simulink model "mo_hinh_dwt_wiener"  (R2026b)
settings: Solver=FixedStepDiscrete  StopTime=5.2480000000000002  FixedStep=6.2500000000000001e-05
InitFcn:
  | model = bdroot;
  | roleMatches=find_system(model,'LookUnderMasks','all','FollowLinks','off','IncludeCommented','on','Tag','WaveletDSP:source');
  | assert(numel(roleMatches)==1,'WaveletDSP:Role','Thiếu hoặc trùng định danh nội bộ: source. Không cần khôi phục tên hiển thị.');
  | source=get_param(roleMatches{1},'Handle');
  | roleMatches=find_system(model,'LookUnderMasks','all','FollowLinks','off','IncludeCommented','on','Tag','WaveletDSP:clean');
  | assert(numel(roleMatches)==1,'WaveletDSP:Role','Thiếu hoặc trùng định danh nội bộ: clean. Không cần khôi phục tên hiển thị.');
  | cleanSource=get_param(roleMatches{1},'Handle');
  | roleMatches=find_system(model,'LookUnderMasks','all','FollowLinks','off','IncludeCommented','on','Tag','WaveletDSP:sink');
  | assert(numel(roleMatches)==1,'WaveletDSP:Role','Thiếu hoặc trùng định danh nội bộ: sink. Không cần khôi phục tên hiển thị.');
  | sink=get_param(roleMatches{1},'Handle');
  | roleMatches=find_system(model,'LookUnderMasks','all','FollowLinks','off','IncludeCommented','on','Tag','WaveletDSP:filter');
  | assert(numel(roleMatches)==1,'WaveletDSP:Role','Thiếu hoặc trùng định danh nội bộ: filter. Không cần khôi phục tên hiển thị.');
  | filterBlock=get_param(roleMatches{1},'Handle');
  | roleMatches=find_system(model,'LookUnderMasks','all','FollowLinks','off','IncludeCommented','on','Tag','WaveletDSP:reference_sync');
  | assert(numel(roleMatches)==1,'WaveletDSP:Role','Thiếu hoặc trùng định danh nội bộ: reference_sync. Không cần khôi phục tên hiển thị.');
  | referenceSync=get_param(roleMatches{1},'Handle');
  | roleMatches=find_system(model,'LookUnderMasks','all','FollowLinks','off','IncludeCommented','on','Tag','WaveletDSP:noisy_sync');
  | assert(numel(roleMatches)==1,'WaveletDSP:Role','Thiếu hoặc trùng định danh nội bộ: noisy_sync. Không cần khôi phục tên hiển thị.');
  | noisySync=get_param(roleMatches{1},'Handle');
  | workspace = get_param(model,'ModelWorkspace');
  | assignin(workspace,'Export_Complete',false);
  | inputFile = get_param(source,'inputFilename');
  | inputInfo = audioinfo(inputFile);
  | assert(inputInfo.NumChannels==1,'Chỉ hỗ trợ âm thanh một kênh.');
  | useClean = strcmp(get_param(filterBlock,'Use_Clean'),'1');
  | cleanFile = get_param(cleanSource,'inputFilename');
  | if useClean && strcmp(get_param(filterBlock,'Auto_Clean'),'1')
  |     [inputFolder,inputStem] = fileparts(inputFile);
  |     recordId = regexp(inputStem,'^(speech_\d+)_','tokens','once');
  |     assert(~isempty(recordId),'Không tìm được âm thanh sạch; tắt ghép tệp tự động và chọn tệp tham chiếu trực tiếp.');
  |     cleanFile = fullfile(fileparts(fileparts(inputFolder)),'clean',[recordId{1} '.wav']);
  | end
  | frameSize = str2double(get_param(source,'SamplesPerFrame'));
  | assert(isfinite(frameSize) && frameSize>0 && mod(frameSize,128)==0,'Số mẫu mỗi khung âm thanh có nhiễu phải là bội dương của 128.');
  | if useClean
  |     cleanInfo = audioinfo(cleanFile);
  |     assert(cleanInfo.SampleRate==inputInfo.SampleRate && cleanInfo.TotalSamples==inputInfo.TotalSamples && cleanInfo.NumChannels==1,'Âm thanh sạch/noisy must match sample rate and length.');
  |     if ~strcmp(get_param(filterBlock,'Auto_Frame'),'1')
  |         assert(str2double(get_param(cleanSource,'SamplesPerFrame'))==frameSize,'Âm thanh sạch/Noisy frame sizes differ. Set them explicitly or enable Auto_Frame.');
  |     end
  | end
  | levels = [1 2 3 4 5 6 7 7];
  | powerWindow = str2double(get_param(filterBlock,'Win_Pow'));
  | smoothWindow = str2double(get_param(filterBlock,'Win_Smooth'));
  | powerLengths = max(1,round(powerWindow*inputInfo.SampleRate./2.^levels));
  | smoothLengths = max(1,round(smoothWindow*inputInfo.SampleRate./2.^levels));
  | bandDelays = floor((powerLengths-1)/2)+floor((smoothLengths-1)/2);
  | totalDelay = 29*(2^7-1)+128*ceil(max(bandDelays.*2.^levels)/128);
  | frameCount = ceil((inputInfo.TotalSamples+totalDelay)/frameSize);
  | requiredStop = (frameCount-1)*frameSize/inputInfo.SampleRate;
  | autoRun = strcmp(get_param(filterBlock,'Auto_Run'),'1');
  | if ~autoRun
  |     assert(strcmp(get_param(model,'Solver'),'FixedStepDiscrete'),'Chọn bộ giải rời rạc bước cố định hoặc bật tự tính thời gian mô phỏng.');
  |     stepValue = slResolve(get_param(model,'FixedStep'),model);
  |     stopValue = slResolve(get_param(model,'StopTime'),model);
  |     assert(isscalar(stepValue) && isfinite(stepValue) && stepValue>0 && stepValue<=1/inputInfo.SampleRate && abs((1/inputInfo.SampleRate)/stepValue-round((1/inputInfo.SampleRate)/stepValue))<1e-8,'Bước mô phỏng phải chia hết chu kỳ lấy mẫu; chỉnh bước hoặc bật tự tính thời gian.');
  |     assert(isscalar(stopValue) && isfinite(stopValue) && stopValue>=requiredStop,'Thời gian dừng quá ngắn hoặc vô hạn; đặt thời gian hữu hạn đủ dài hoặc bật tự tính thời gian.');
  | end
  | configuredOutput = get_param(sink,'outputFilename');
  | assert(~strcmp(inputFile,configuredOutput) && ~strcmp(cleanFile,configuredOutput),'Tệp đầu ra không được trùng tệp đầu vào.');
  | [outputFolder,outputStem,outputExtension] = fileparts(configuredOutput);
  | if isempty(outputFolder), outputFolder=pwd; end
  | if ~isfolder(outputFolder), mkdir(outputFolder); end
  | runtimeOutput = configuredOutput;
  | if isfile(runtimeOutput)
  |     runtimeOutput = fullfile(outputFolder,[outputStem '_' char(datetime('now','Format','yyyyMMdd_HHmmss_SSS')) outputExtension]);
  |     assert(~isfile(runtimeOutput),'Trùng tên tệp đầu ra; chọn tên khác và chạy lại.');
  | end
  | restoreSettings = struct('CleanFile',get_param(cleanSource,'inputFilename'),'CleanFrame',get_param(cleanSource,'SamplesPerFrame'),'CleanCommented',get_param(cleanSource,'Commented'),'OutputFile',configuredOutput,'SolverType',get_param(model,'SolverType'),'Solver',get_param(model,'Solver'),'FixedStep',get_param(model,'FixedStep'),'StopTime',get_param(model,'StopTime'));
  | assignin(workspace,'Run_Restore_Settings',restoreSettings);
  | assignin(workspace,'Last_Output_File',runtimeOutput);
  | assignin(workspace,'Total_Delay',totalDelay);
  | for syncBlock=[referenceSync noisySync]
  |     countText=sprintf('%.0f',totalDelay);
  |     if ~strcmp(get_param(syncBlock,'Sample_Count'),countText), set_param(syncBlock,'Sample_Count',countText); end
  | end
  | assignin(workspace,'Valid_Samples',inputInfo.TotalSamples);
  | assignin(workspace,'Audio_Fs',inputInfo.SampleRate);
  | assignin(workspace,'Frame_Size',frameSize);
  | assignin(workspace,'Reference_Available',double(useClean));
  | assignin(workspace,'Run_Clean_File',cleanFile);
  | if useClean
  |     set_param(cleanSource,'inputFilename',cleanFile,'Commented','off');
  |     referenceSource = cleanSource;
  | else
  |     set_param(cleanSource,'inputFilename',inputFile,'Commented','on');
  |     referenceSource = source;
  | end
  | if strcmp(get_param(filterBlock,'Auto_Frame'),'1'), set_param(cleanSource,'SamplesPerFrame',num2str(frameSize)); end
  | referencePorts = get_param(referenceSync,'PortHandles');
  | referenceLine = get_param(referencePorts.Inport(1),'Line');
  | if referenceLine~=-1
  |     oldSource = get_param(get_param(get_param(referenceLine,'SrcPortHandle'),'Parent'),'Handle');
  |     if oldSource~=referenceSource
  |         delete_line(referenceLine);
  |         sourcePorts=get_param(referenceSource,'PortHandles');
  |         add_line(model,sourcePorts.Outport(1),referencePorts.Inport(1),'autorouting','on');
  |     end
  | else
  |     sourcePorts=get_param(referenceSource,'PortHandles');
  |     add_line(model,sourcePorts.Outport(1),referencePorts.Inport(1),'autorouting','on');
  | end
  | if autoRun
  |     set_param(model,'SolverType','Fixed-step','Solver','FixedStepDiscrete','FixedStep',sprintf('%.17g',1/inputInfo.SampleRate),'StopTime',sprintf('%.17g',requiredStop));
  | end
  | set_param(sink,'outputFilename',runtimeOutput);
  | fprintf('Có tham chiếu=%d. Tệp đầu ra thực tế: %s\n',useClean,runtimeOutput);
StopFcn:
  | model = bdroot;
  | workspace = get_param(model,'ModelWorkspace');
  | roleMatches=find_system(model,'LookUnderMasks','all','FollowLinks','off','IncludeCommented','on','Tag','WaveletDSP:sink');
  | assert(numel(roleMatches)==1,'WaveletDSP:Role','Thiếu hoặc trùng định danh nội bộ: sink. Không cần khôi phục tên hiển thị.');
  | sink=get_param(roleMatches{1},'Handle');
  | roleMatches=find_system(model,'LookUnderMasks','all','FollowLinks','off','IncludeCommented','on','Tag','WaveletDSP:clean');
  | assert(numel(roleMatches)==1,'WaveletDSP:Role','Thiếu hoặc trùng định danh nội bộ: clean. Không cần khôi phục tên hiển thị.');
  | cleanSource=get_param(roleMatches{1},'Handle');
  | outputFile = evalin(workspace,'Last_Output_File');
  | restoreSettings = evalin(workspace,'Run_Restore_Settings');
  | set_param(sink,'outputFilename',restoreSettings.OutputFile);
  | set_param(cleanSource,'inputFilename',restoreSettings.CleanFile,'Commented',restoreSettings.CleanCommented);
  | [outputAudio,outputRate] = audioread(outputFile);
  | delaySamples = evalin(workspace,'Total_Delay');
  | validSamples = evalin(workspace,'Valid_Samples');
  | assert(size(outputAudio,1)>=delaySamples+validSamples,'Mô phỏng dừng sớm: đầu ra chưa đủ mẫu; tệp thô được giữ lại.');
  | outputAudio = outputAudio(delaySamples+(1:validSamples),:);
  | audiowrite(outputFile,outputAudio,outputRate,'BitsPerSample',24);
  | assignin(workspace,'Export_Complete',true);
  | fprintf('Đã xuất âm thanh và giữ thiết lập. Tệp âm thanh: %s\n',outputFile);
model workspace (MAT data in the model file):
  Audio_Fs = 16000
  Export_Complete = 1
  Frame_Size = 1024
  Last_Output_File = '/home/alberttochiro/Documents/Codex/PRJ/WaveletDSP/results/denoised_output_20261108_091202_407.wav'
  Reference_Available = 1
  Run_Clean_File = '/home/alberttochiro/Documents/Codex/PRJ/WaveletDSP/data_DSP_speech/clean/speech_004.wav'
  Run_Restore_Settings.CleanFile = '/home/alberttochiro/Documents/Codex/PRJ/WaveletDSP/data_DSP_speech/clean/speech_004.wav'
  Run_Restore_Settings.CleanFrame = '1024'
  Run_Restore_Settings.CleanCommented = 'off'
  Run_Restore_Settings.OutputFile = '/home/alberttochiro/Documents/Codex/PRJ/WaveletDSP/results/denoised_output.wav'
  Run_Restore_Settings.SolverType = 'Fixed-step'
  Run_Restore_Settings.Solver = 'FixedStepDiscrete'
  Run_Restore_Settings.FixedStep = '6.2500000000000001e-05'
  Run_Restore_Settings.StopTime = '5.2480000000000002'
  Total_Delay = 4579
  Valid_Samples = 79500
undefined symbols (not defined in the file or in its folder): dspblkCoreblockFVToolHelper, gcbh, Pn_1, Pn_2, Pn_3, Pn_4, Pn_5, Pn_6, Pn_7, Pn_8
libraries: dspvision x3, dspmlti4 x2, simulink x2
(part 1 of 2)
settings Model: Creator=alberttochiro  LastModifiedBy=alberttochiro

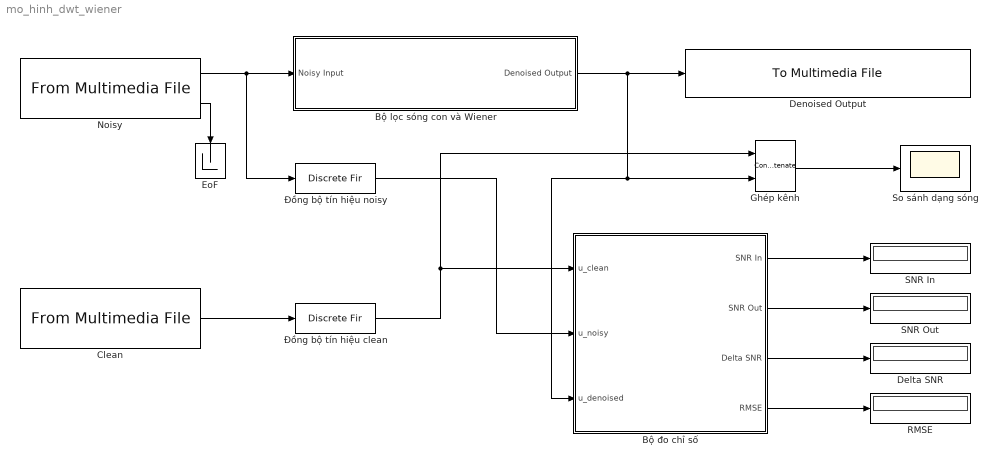
== system mo_hinh_dwt_wiener ==
  Bộ lọc sóng con và Wiener : Subsystem  Tag=WaveletDSP:filter  mask(Bo Loc Wavelet DWT Wiener Full Native){Noise_Sec=0.25, Win_Pow=0.064, Win_Smooth=0.040, Gain_Floor=0.05, Auto_Clean=1, Noise_Auto=1, Noise_Powers=[0.000004 0.000008 0.000014 0.000025 0.000055 0.000108 0.000112 0.002000], Use_Clean=1, Clean_File=/home/alberttochiro/Documents/Codex/PRJ/WaveletDSP/data_DSP_speech/clean/speech_003.wav, Noise_Start_Auto=1, Noise_Start=0, Auto_Run=0, Auto_Frame=0, Noise_Power_1=4e-06, Noise_Power_2=8e-06, Noise_Power_3=1.4e-05, Noise_Power_4=2.5e-05, Noise_Power_5=5.5e-05, Noise_Power_6=0.000108, Noise_Power_7=0.000112, Noise_Power_8=0.002}
      mask prompts: Noise_Sec "Độ dài mẫu nhiễu (giây)"; Win_Pow "Cửa sổ tính công suất (giây)"; Win_Smooth "Cửa sổ làm mượt hệ số khuếch đại (giây)"; Gain_Floor "Hệ số khuếch đại tối thiểu (từ 0 đến 1)"; Auto_Clean "Tự ghép tệp âm thanh sạch cùng bản ghi (1 là bật, 0 là tắt)"; Noise_Auto "Tự ước lượng công suất nhiễu (1 là bật, 0 là nhập tay)"; Noise_Powers "Công suất nhiễu tám dải khi nhập tay"; Use_Clean "Dùng âm thanh sạch để đánh giá (1 là có, 0 là không)"; Clean_File "Đường dẫn tham chiếu cũ (không sử dụng)"; Noise_Start_Auto "Tự bỏ đoạn đầu hằng khi lấy mẫu nhiễu (1 là tự động, 0 là chọn tay)"; Noise_Start "Thời điểm bắt đầu lấy mẫu nhiễu thủ công (giây)"; Auto_Run "Tự tính bước và thời gian mô phỏng (1 là bật, 0 là giữ thiết lập)"; Auto_Frame "Tự đồng bộ kích thước khung tham chiếu (1 là bật, 0 là kiểm tra)"; Noise_Power_1 "Công suất nhiễu dải 1 khi nhập tay"; Noise_Power_2 "Công suất nhiễu dải 2 khi nhập tay"; Noise_Power_3 "Công suất nhiễu dải 3 khi nhập tay"; Noise_Power_4 "Công suất nhiễu dải 4 khi nhập tay"; Noise_Power_5 "Công suất nhiễu dải 5 khi nhập tay"; Noise_Power_6 "Công suất nhiễu dải 6 khi nhập tay"; Noise_Power_7 "Công suất nhiễu dải 7 khi nhập tay"; Noise_Power_8 "Công suất nhiễu dải 8 khi nhập tay"
      mask help:
      | Bộ lọc phân rã sóng con bảy mức kết hợp Wiener.
      | Các khối xử lý tín hiệu giữ nguyên công thức. Ước lượng nhiễu vẫn nằm trong phần khởi tạo mặt nạ.
      | Không cần chạy tệp lệnh bên ngoài. Đoạn lấy mẫu nhiễu phải chỉ chứa tiếng nền, không có lời nói.
      mask init:
      | validateattributes(Noise_Power_1,{'double'},{'scalar','real','finite','nonnegative'});
      | validateattributes(Noise_Power_2,{'double'},{'scalar','real','finite','nonnegative'});
      | validateattributes(Noise_Power_3,{'double'},{'scalar','real','finite','nonnegative'});
      | validateattributes(Noise_Power_4,{'double'},{'scalar','real','finite','nonnegative'});
      | validateattributes(Noise_Power_5,{'double'},{'scalar','real','finite','nonnegative'});
      | validateattributes(Noise_Power_6,{'double'},{'scalar','real','finite','nonnegative'});
      | validateattributes(Noise_Power_7,{'double'},{'scalar','real','finite','nonnegative'});
      | validateattributes(Noise_Power_8,{'double'},{'scalar','real','finite','nonnegative'});
      | roleMatches=find_system(bdroot,'LookUnderMasks','all','FollowLinks','off','IncludeCommented','on','Tag','WaveletDSP:source');
      | assert(numel(roleMatches)==1,'WaveletDSP:Role','Thiếu hoặc trùng định danh nội bộ: source. Không cần khôi phục tên hiển thị.');
      | audioSource=get_param(roleMatches{1},'Handle');
      | inFile = get_param(audioSource,'inputFilename');
      | inputInfo = audioinfo(inFile);
      | Fs = inputInfo.SampleRate;
      | validateattributes(Win_Pow, {'double'}, {'scalar','positive','finite'});
      | validateattributes(Win_Smooth, {'double'}, {'scalar','positive','finite'});
      | validateattributes(Gain_Floor, {'double'}, {'scalar','>=',0,'<=',1});
      | wname = 'coif5';
      | lev = 7;
      | if Noise_Auto == 1
      |         [x_calib, Fs_calib] = audioread(inFile);
      | validateattributes(Noise_Sec,{'double'},{'scalar','real','finite','positive'});
      | validateattributes(Noise_Start,{'double'},{'scalar','real','finite','nonnegative'});
      | validateattributes(Noise_Start_Auto,{'double'},{'scalar','binary'});
      | assert(size(x_calib,2)==1 && all(isfinite(x_calib(:))), 'WaveletDSP:InvalidNoiseProfile', 'Mẫu nhiễu cần âm thanh một kênh có giá trị hữu hạn.');
      | N_n = floor(Noise_Sec*Fs_calib);
      | Startup_Skipped_Samples = 0;
      | if Noise_Start_Auto==1
      |     firstChanged = find(x_calib~=x_calib(1),1,'first');
      |     assert(~isempty(firstChanged), 'WaveletDSP:ConstantRecording', 'Toàn bộ bản ghi có giá trị hằng. Hãy ghi tiếng nền trước khi nói hoặc nhập công suất nhiễu thủ công.');
      |     if firstChanged-1>=ceil(0.010*Fs_calib)
      |         Startup_Skipped_Samples = firstChanged-1;
      |     end
      |     Noise_Profile_Start_Sample = Startup_Skipped_Samples+1;
      | else
      |     Noise_Profile_Start_Sample = floor(Noise_Start*Fs_calib)+1;
      | end
      | Noise_Profile_End_Sample = Noise_Profile_Start_Sample+N_n-1;
      | assert(N_n>=1024 && Noise_Profile_End_Sample<=numel(x_calib), 'WaveletDSP:InvalidNoiseProfile', 'Mẫu nhiễu cần ít nhất 1024 mẫu và không vượt cuối tệp; giảm độ dài hoặc chọn lại thời điểm bắt đầu.');
      | noiseProfile = x_calib(Noise_Profile_Start_Sample:Noise_Profile_End_Sample);
      | assert(var(noiseProfile,1)>eps(max(abs(noiseProfile)))^2, 'WaveletDSP:ConstantNoiseProfile', 'Mẫu nhiễu được chọn có giá trị hằng hoặc gần hằng ở mức sai số số học. Bật tự bỏ đoạn đầu hằng hoặc chọn lại đoạn chỉ có tiếng nền.');
      | fprintf('Mẫu nhiễu: bắt đầu=%.9f giây, độ dài=%.9f giây, bỏ đoạn đầu hằng=%d mẫu. Chức năng này không phát hiện tiếng nói.\n', (Noise_Profile_Start_Sample-1)/Fs_calib,N_n/Fs_calib,Startup_Skipped_Samples);
      | [C_n, L_n] = wavedec(noiseProfile, lev, wname, 'Mode', 'sym');
      | Pn_vec = zeros(1, 8);
      |         for k = 1:7
      |             Pn_vec(k) = var(detcoef(C_n, L_n, k), 1);
      |         end
      |         Pn_vec(8) = var(appcoef(C_n, L_n, wname, 7), 1);
      | else
      |     Pn_vec = [Noise_Power_1 Noise_Power_2 Noise_Power_3 Noise_Power_4 Noise_Power_5 Noise_Power_6 Noise_Power_7 Noise_Power_8];
      | end
      | validateattributes(Pn_vec, {'double'}, {'vector','numel',8,'nonnegative','finite'});
      | levels = [1, 2, 3, 4, 5, 6, 7, 7];
      | delays_tree = [1827, 899, 435, 203, 87, 29, 0, 0];
      | window_power = max(1, round(Win_Pow*Fs./2.^levels));
      | window_smooth = max(1, round(Win_Smooth*Fs./2.^levels));
      | sync_delays = floor((window_power-1)/2)+floor((window_smooth-1)/2);
      | common_delay = 128*ceil(max(sync_delays.*2.^levels)/128);
      | delays_tree = delays_tree+(common_delay-sync_delays.*2.^levels)./2.^levels;
      | for k = 1:8
      |     Fs_k = Fs / (2^levels(k));
      |     w_pow_k = max(1, round(Win_Pow * Fs_k));
      |     w_sm_k = max(1, round(Win_Smooth * Fs_k));
      |     d_sync_k = floor((w_pow_k - 1)/2) + floor((w_sm_k - 1)/2);
      |     eval(sprintf('b_pow_%d = ones(1, %d)/%d;', k, w_pow_k, w_pow_k));
      |     eval(sprintf('b_sm_%d = ones(1, %d)/%d;', k, w_sm_k, w_sm_k));
      |     eval(sprintf('b_sync_%d = [zeros(1, %d), 1];', k, d_sync_k));
      |     eval(sprintf('b_tree_%d = [zeros(1, %d), 1];', k, delays_tree(k)));
      |     eval(sprintf('Pn_%d = %.12e;', k, Pn_vec(k)));
      | end
      | 
      | numericInterfaceVersion='WaveletDSP:NumericInterface';
      | for bandIndex=1:8
      |     counts=[sync_delays(bandIndex) window_power(bandIndex) window_smooth(bandIndex) delays_tree(bandIndex)];
      |     kinds={'sync','pow','sm','tree'};
      |     for kindIndex=1:4
      |         roleName=sprintf('WaveletDSP:%s_%d',kinds{kindIndex},bandIndex);
      |         matches=find_system(bdroot,'LookUnderMasks','all','FollowLinks','off','IncludeCommented','on','Tag',roleName);
      |         assert(numel(matches)==1,'WaveletDSP:Role','Thiếu hoặc trùng định danh nội bộ: %s.',roleName);
      |         countText=sprintf('%.0f',counts(kindIndex));
      |         if ~strcmp(get_param(matches{1},'Sample_Count'),countText), set_param(matches{1},'Sample_Count',countText); end
      |     end
      | end
  Bộ đo chỉ số : Subsystem
  Clean : dspvision/From Multimedia File  Tag=WaveletDSP:clean  inputFilename=/home/alberttochiro/Documents/Codex/PRJ/WaveletDSP/data_DSP_speech/clean/speech_004.wav  readRange=[1 Inf]  loop=on  numPlays=1  outputStreams=Audio only  videoDataType=single  audioDataType=double  inheritSampleTime=on  userDefinedSampleTime=1/30  noAudioOutput=off  isIntensityVideo=off  fourcc=RGB  colorVideoFormat=One multidimensional signal  outputEOF=off  dataOrg=Column-major  audioFrameSize=1024  computeAudioFrameSize=off  outSamplingMode=Sample based
      settings: LibrarySourceBlock=dspsrcs4/From Multimedia File
  Delta SNR : Display
  Denoised Output : dspvision/To Multimedia File  Tag=WaveletDSP:sink  outputFilename=/home/alberttochiro/Documents/Codex/PRJ/WaveletDSP/results/denoised_output.wav  streamSelection=Audio only  videoCompressor=None (uncompressed)  audioCompressor=None (uncompressed)  imagePorts=One multidimensional signal  fileType=WAV  audioDatatype=24-bit integer  fourcc=RGB  audioBitRate=128  audioQuality=75  videoQuality=75  mj2000CompFactor=10
  EoF : Terminator
  Ghép kênh : Concatenate  Mode=Multidimensional array  ConcatenateDimension=2
  Noisy : dspvision/From Multimedia File  Tag=WaveletDSP:source  inputFilename=/home/alberttochiro/Documents/Codex/PRJ/WaveletDSP/data_DSP_speech/noisy/white_10db/speech_004_white_10dB.wav  readRange=[1 Inf]  loop=on  numPlays=1  outputStreams=Audio only  videoDataType=single  audioDataType=double  inheritSampleTime=on  userDefinedSampleTime=1/30  noAudioOutput=off  isIntensityVideo=off  fourcc=RGB  colorVideoFormat=One multidimensional signal  outputEOF=on  dataOrg=Column-major  audioFrameSize=1024  computeAudioFrameSize=off  outSamplingMode=Sample based
      settings: LibrarySourceBlock=dspsrcs4/From Multimedia File
  RMSE : Display
  SNR In : Display
  SNR Out : Display
  So sánh dạng sóng : Scope
      settings: TimeUnits=Metric (based on Time Span)  ActiveDisplayYMinimum=-0.42486149114836624  ActiveDisplayYMaximum=0.39931183525403668  YLabel=Amplitude
  Đồng bộ tín hiệu clean : DiscreteFir  Tag=WaveletDSP:reference_sync  LoadFcn=dspblkCoreblockFVToolHelper(gcbh,'load');  Coefficients=[zeros(1,Sample_Count) 1]  InputProcessing=Columns as channels (frame based)  mask{Sample_Count=4579}
      mask prompts: Sample_Count "Số mẫu đồng bộ (tự tính từ cấu trúc và thiết lập bộ lọc)"
      mask help: Đồng bộ tín hiệu theo số mẫu. Giá trị được tính tự động để giữ nguyên phép lọc; không cần nhập dãy hệ số.
      mask init:
      | validateattributes(Sample_Count,{'double'},{'scalar','integer','finite','>=',0});
      settings: CopyFcn=dspblkCoreblockFVToolHelper(gcbh,'copy');  DeleteFcn=dspblkCoreblockFVToolHelper(gcbh,'close');  ModelCloseFcn=dspblkCoreblockFVToolHelper(gcbh,'close');  PreSaveFcn=dspblkCoreblockFVToolHelper(gcbh,'presave');  PostSaveFcn=dspblkCoreblockFVToolHelper(gcbh,'postsave');  CloseFcn=dspblkCoreblockFVToolHelper(gcbh,'close');
  Đồng bộ tín hiệu noisy : DiscreteFir  Tag=WaveletDSP:noisy_sync  LoadFcn=dspblkCoreblockFVToolHelper(gcbh,'load');  Coefficients=[zeros(1,Sample_Count) 1]  InputProcessing=Columns as channels (frame based)  mask{Sample_Count=4579}
      mask prompts: Sample_Count "Số mẫu đồng bộ (tự tính từ cấu trúc và thiết lập bộ lọc)"
      mask help: Đồng bộ tín hiệu theo số mẫu. Giá trị được tính tự động để giữ nguyên phép lọc; không cần nhập dãy hệ số.
      mask init:
      | validateattributes(Sample_Count,{'double'},{'scalar','integer','finite','>=',0});
      settings: CopyFcn=dspblkCoreblockFVToolHelper(gcbh,'copy');  DeleteFcn=dspblkCoreblockFVToolHelper(gcbh,'close');  ModelCloseFcn=dspblkCoreblockFVToolHelper(gcbh,'close');  PreSaveFcn=dspblkCoreblockFVToolHelper(gcbh,'presave');  PostSaveFcn=dspblkCoreblockFVToolHelper(gcbh,'postsave');  CloseFcn=dspblkCoreblockFVToolHelper(gcbh,'close');
  wires:
  Noisy/2 -> EoF/1
  Noisy/1 -> Bộ lọc sóng con và Wiener/1(Noisy Input), Đồng bộ tín hiệu noisy/1
  Đồng bộ tín hiệu noisy/1 -> Bộ đo chỉ số/2(u_noisy)
  Bộ lọc sóng con và Wiener/1(Denoised Output) -> Bộ đo chỉ số/3(u_denoised), Ghép kênh/2, Denoised Output/1
  Đồng bộ tín hiệu clean/1 -> Ghép kênh/1, Bộ đo chỉ số/1(u_clean)
  Ghép kênh/1 -> So sánh dạng sóng/1
  Bộ đo chỉ số/1(SNR In) -> SNR In/1
  Bộ đo chỉ số/2(SNR Out) -> SNR Out/1
  Bộ đo chỉ số/3(Delta SNR) -> Delta SNR/1
  Bộ đo chỉ số/4(RMSE) -> RMSE/1
  Clean/1 -> Đồng bộ tín hiệu clean/1

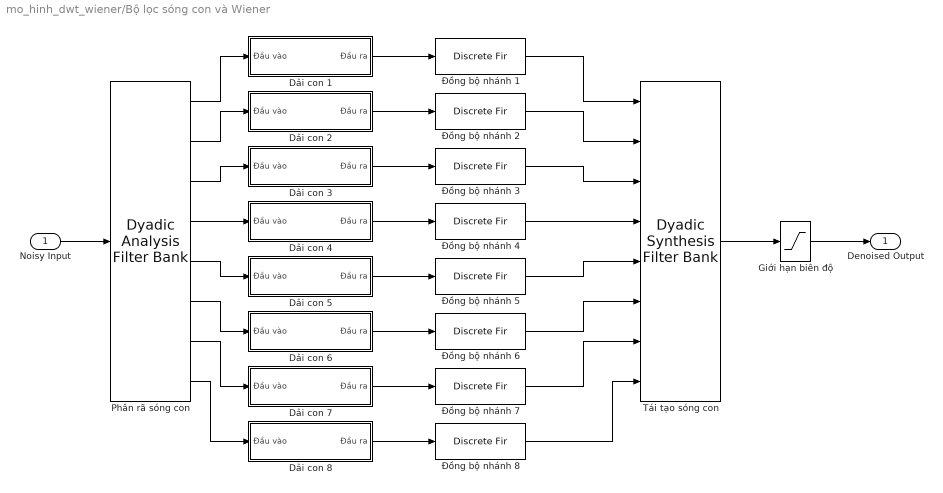
== system mo_hinh_dwt_wiener/Bộ lọc sóng con và Wiener ==
  Noisy Input : Inport
  Dải con 1 : Subsystem  Tag=WaveletDSP:band_1
  Dải con 2 : Subsystem  Tag=WaveletDSP:band_2
  Dải con 3 : Subsystem  Tag=WaveletDSP:band_3
  Dải con 4 : Subsystem  Tag=WaveletDSP:band_4
  Dải con 5 : Subsystem  Tag=WaveletDSP:band_5
  Dải con 6 : Subsystem  Tag=WaveletDSP:band_6
  Dải con 7 : Subsystem  Tag=WaveletDSP:band_7
  Dải con 8 : Subsystem  Tag=WaveletDSP:band_8
  Giới hạn biên độ : Saturate  UpperLimit=1.0  LowerLimit=-1.0
  Phân rã sóng con : dspmlti4/Dyadic Analysis Filter Bank  Wname=Coiflets  OrdRec_ordDec=[1 / 1]  Order=5  LPF="[0.0352   -0.0854   -0.1350   0.4599   0.8069   0.3327]"  HPF="[-0.3327    0.8069   -0.4599   -0.1350    0.0854    0.0352]"  NumLevels=7  tree=Asymmetric  Output=Multiple ports  OutputFrames=off
      settings: LibrarySourceBlock=dspxfrm3/DWT
  Tái tạo sóng con : dspmlti4/Dyadic Synthesis Filter Bank  Wname=Coiflets  OrdRec_ordDec=[1 / 1]  Order=5  LPF="[0.3327    0.8069    0.4599   -0.1350   -0.0854    0.0352]"  HPF="[0.0352    0.0854   -0.1350   -0.4599    0.8069   -0.3327]"  NumLevels=7  tree=Asymmetric  Input=Multiple ports  OutputFrames=off
      settings: LibrarySourceBlock=dspxfrm3/IDWT
  Đồng bộ nhánh 1 : DiscreteFir  Tag=WaveletDSP:tree_1  LoadFcn=dspblkCoreblockFVToolHelper(gcbh,'load');  Coefficients=[zeros(1,Sample_Count) 1]  InputProcessing=Columns as channels (frame based)  mask{Sample_Count=1861}
      mask prompts: Sample_Count "Số mẫu đồng bộ (tự tính từ cấu trúc và thiết lập bộ lọc)"
      mask help: Đồng bộ tín hiệu theo số mẫu. Giá trị được tính tự động để giữ nguyên phép lọc; không cần nhập dãy hệ số.
      mask init:
      | validateattributes(Sample_Count,{'double'},{'scalar','integer','finite','>=',0});
      settings: CopyFcn=dspblkCoreblockFVToolHelper(gcbh,'copy');  DeleteFcn=dspblkCoreblockFVToolHelper(gcbh,'close');  ModelCloseFcn=dspblkCoreblockFVToolHelper(gcbh,'close');  PreSaveFcn=dspblkCoreblockFVToolHelper(gcbh,'presave');  PostSaveFcn=dspblkCoreblockFVToolHelper(gcbh,'postsave');  CloseFcn=dspblkCoreblockFVToolHelper(gcbh,'close');
  Đồng bộ nhánh 2 : DiscreteFir  Tag=WaveletDSP:tree_2  LoadFcn=dspblkCoreblockFVToolHelper(gcbh,'load');  Coefficients=[zeros(1,Sample_Count) 1]  InputProcessing=Columns as channels (frame based)  mask{Sample_Count=917}
      mask prompts: Sample_Count "Số mẫu đồng bộ (tự tính từ cấu trúc và thiết lập bộ lọc)"
      mask help: Đồng bộ tín hiệu theo số mẫu. Giá trị được tính tự động để giữ nguyên phép lọc; không cần nhập dãy hệ số.
      mask init:
      | validateattributes(Sample_Count,{'double'},{'scalar','integer','finite','>=',0});
      settings: CopyFcn=dspblkCoreblockFVToolHelper(gcbh,'copy');  DeleteFcn=dspblkCoreblockFVToolHelper(gcbh,'close');  ModelCloseFcn=dspblkCoreblockFVToolHelper(gcbh,'close');  PreSaveFcn=dspblkCoreblockFVToolHelper(gcbh,'presave');  PostSaveFcn=dspblkCoreblockFVToolHelper(gcbh,'postsave');  CloseFcn=dspblkCoreblockFVToolHelper(gcbh,'close');
  Đồng bộ nhánh 3 : DiscreteFir  Tag=WaveletDSP:tree_3  Coefficients=[zeros(1,Sample_Count) 1]  InputProcessing=Columns as channels (frame based)  mask{Sample_Count=445}
      mask prompts: Sample_Count "Số mẫu đồng bộ (tự tính từ cấu trúc và thiết lập bộ lọc)"
      mask help: Đồng bộ tín hiệu theo số mẫu. Giá trị được tính tự động để giữ nguyên phép lọc; không cần nhập dãy hệ số.
      mask init:
      | validateattributes(Sample_Count,{'double'},{'scalar','integer','finite','>=',0});
  Đồng bộ nhánh 4 : DiscreteFir  Tag=WaveletDSP:tree_4  Coefficients=[zeros(1,Sample_Count) 1]  InputProcessing=Columns as channels (frame based)  mask{Sample_Count=209}
      mask prompts: Sample_Count "Số mẫu đồng bộ (tự tính từ cấu trúc và thiết lập bộ lọc)"
      mask help: Đồng bộ tín hiệu theo số mẫu. Giá trị được tính tự động để giữ nguyên phép lọc; không cần nhập dãy hệ số.
      mask init:
      | validateattributes(Sample_Count,{'double'},{'scalar','integer','finite','>=',0});
  Đồng bộ nhánh 5 : DiscreteFir  Tag=WaveletDSP:tree_5  LoadFcn=dspblkCoreblockFVToolHelper(gcbh,'load');  Coefficients=[zeros(1,Sample_Count) 1]  InputProcessing=Columns as channels (frame based)  mask{Sample_Count=91}
      mask prompts: Sample_Count "Số mẫu đồng bộ (tự tính từ cấu trúc và thiết lập bộ lọc)"
      mask help: Đồng bộ tín hiệu theo số mẫu. Giá trị được tính tự động để giữ nguyên phép lọc; không cần nhập dãy hệ số.
      mask init:
      | validateattributes(Sample_Count,{'double'},{'scalar','integer','finite','>=',0});
      settings: CopyFcn=dspblkCoreblockFVToolHelper(gcbh,'copy');  DeleteFcn=dspblkCoreblockFVToolHelper(gcbh,'close');  ModelCloseFcn=dspblkCoreblockFVToolHelper(gcbh,'close');  PreSaveFcn=dspblkCoreblockFVToolHelper(gcbh,'presave');  PostSaveFcn=dspblkCoreblockFVToolHelper(gcbh,'postsave');  CloseFcn=dspblkCoreblockFVToolHelper(gcbh,'close');
  Đồng bộ nhánh 6 : DiscreteFir  Tag=WaveletDSP:tree_6  LoadFcn=dspblkCoreblockFVToolHelper(gcbh,'load');  Coefficients=[zeros(1,Sample_Count) 1]  InputProcessing=Columns as channels (frame based)  mask{Sample_Count=32}
      mask prompts: Sample_Count "Số mẫu đồng bộ (tự tính từ cấu trúc và thiết lập bộ lọc)"
      mask help: Đồng bộ tín hiệu theo số mẫu. Giá trị được tính tự động để giữ nguyên phép lọc; không cần nhập dãy hệ số.
      mask init:
      | validateattributes(Sample_Count,{'double'},{'scalar','integer','finite','>=',0});
      settings: CopyFcn=dspblkCoreblockFVToolHelper(gcbh,'copy');  DeleteFcn=dspblkCoreblockFVToolHelper(gcbh,'close');  ModelCloseFcn=dspblkCoreblockFVToolHelper(gcbh,'close');  PreSaveFcn=dspblkCoreblockFVToolHelper(gcbh,'presave');  PostSaveFcn=dspblkCoreblockFVToolHelper(gcbh,'postsave');  CloseFcn=dspblkCoreblockFVToolHelper(gcbh,'close');
  Đồng bộ nhánh 7 : DiscreteFir  Tag=WaveletDSP:tree_7  LoadFcn=dspblkCoreblockFVToolHelper(gcbh,'load');  Coefficients=[zeros(1,Sample_Count) 1]  InputProcessing=Columns as channels (frame based)  mask{Sample_Count=2}
      mask prompts: Sample_Count "Số mẫu đồng bộ (tự tính từ cấu trúc và thiết lập bộ lọc)"
      mask help: Đồng bộ tín hiệu theo số mẫu. Giá trị được tính tự động để giữ nguyên phép lọc; không cần nhập dãy hệ số.
      mask init:
      | validateattributes(Sample_Count,{'double'},{'scalar','integer','finite','>=',0});
      settings: CopyFcn=dspblkCoreblockFVToolHelper(gcbh,'copy');  DeleteFcn=dspblkCoreblockFVToolHelper(gcbh,'close');  ModelCloseFcn=dspblkCoreblockFVToolHelper(gcbh,'close');  PreSaveFcn=dspblkCoreblockFVToolHelper(gcbh,'presave');  PostSaveFcn=dspblkCoreblockFVToolHelper(gcbh,'postsave');  CloseFcn=dspblkCoreblockFVToolHelper(gcbh,'close');
  Đồng bộ nhánh 8 : DiscreteFir  Tag=WaveletDSP:tree_8  LoadFcn=dspblkCoreblockFVToolHelper(gcbh,'load');  Coefficients=[zeros(1,Sample_Count) 1]  InputProcessing=Columns as channels (frame based)  mask{Sample_Count=2}
      mask prompts: Sample_Count "Số mẫu đồng bộ (tự tính từ cấu trúc và thiết lập bộ lọc)"
      mask help: Đồng bộ tín hiệu theo số mẫu. Giá trị được tính tự động để giữ nguyên phép lọc; không cần nhập dãy hệ số.
      mask init:
      | validateattributes(Sample_Count,{'double'},{'scalar','integer','finite','>=',0});
      settings: CopyFcn=dspblkCoreblockFVToolHelper(gcbh,'copy');  DeleteFcn=dspblkCoreblockFVToolHelper(gcbh,'close');  ModelCloseFcn=dspblkCoreblockFVToolHelper(gcbh,'close');  PreSaveFcn=dspblkCoreblockFVToolHelper(gcbh,'presave');  PostSaveFcn=dspblkCoreblockFVToolHelper(gcbh,'postsave');  CloseFcn=dspblkCoreblockFVToolHelper(gcbh,'close');
  Denoised Output : Outport
  wires:
  Noisy Input/1 -> Phân rã sóng con/1
  Phân rã sóng con/1 -> Dải con 1/1(Đầu vào)
  Dải con 1/1(Đầu ra) -> Đồng bộ nhánh 1/1
  Đồng bộ nhánh 1/1 -> Tái tạo sóng con/1
  Phân rã sóng con/2 -> Dải con 2/1(Đầu vào)
  Dải con 2/1(Đầu ra) -> Đồng bộ nhánh 2/1
  Đồng bộ nhánh 2/1 -> Tái tạo sóng con/2
  Phân rã sóng con/3 -> Dải con 3/1(Đầu vào)
  Dải con 3/1(Đầu ra) -> Đồng bộ nhánh 3/1
  Đồng bộ nhánh 3/1 -> Tái tạo sóng con/3
  Phân rã sóng con/4 -> Dải con 4/1(Đầu vào)
  Dải con 4/1(Đầu ra) -> Đồng bộ nhánh 4/1
  Đồng bộ nhánh 4/1 -> Tái tạo sóng con/4
  Phân rã sóng con/5 -> Dải con 5/1(Đầu vào)
  Dải con 5/1(Đầu ra) -> Đồng bộ nhánh 5/1
  Đồng bộ nhánh 5/1 -> Tái tạo sóng con/5
  Phân rã sóng con/6 -> Dải con 6/1(Đầu vào)
  Dải con 6/1(Đầu ra) -> Đồng bộ nhánh 6/1
  Đồng bộ nhánh 6/1 -> Tái tạo sóng con/6
  Phân rã sóng con/7 -> Dải con 7/1(Đầu vào)
  Dải con 7/1(Đầu ra) -> Đồng bộ nhánh 7/1
  Đồng bộ nhánh 7/1 -> Tái tạo sóng con/7
  Phân rã sóng con/8 -> Dải con 8/1(Đầu vào)
  Dải con 8/1(Đầu ra) -> Đồng bộ nhánh 8/1
  Đồng bộ nhánh 8/1 -> Tái tạo sóng con/8
  Tái tạo sóng con/1 -> Giới hạn biên độ/1
  Giới hạn biên độ/1 -> Denoised Output/1

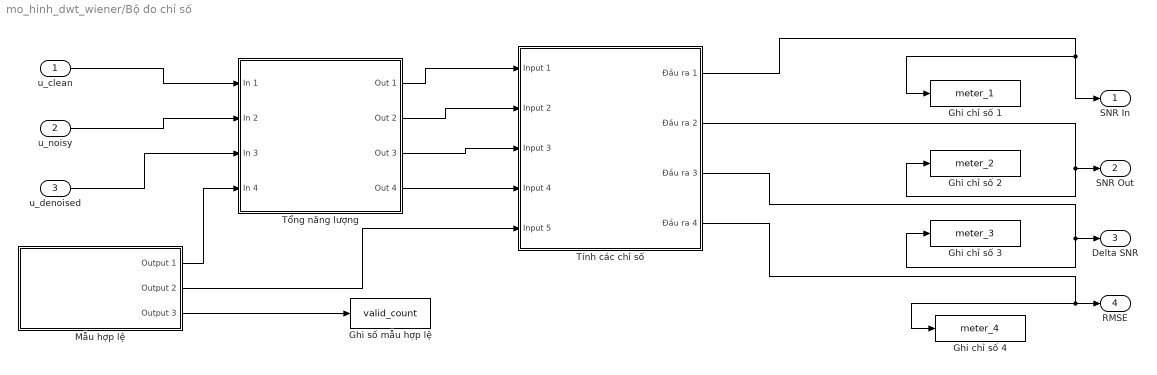
== system mo_hinh_dwt_wiener/Bộ đo chỉ số ==
  u_clean : Inport
  u_noisy : Inport  Port=2
  u_denoised : Inport  Port=3
  Ghi chỉ số 1 : ToWorkspace  VariableName=meter_1  SampleTime=-1
  Ghi chỉ số 2 : ToWorkspace  VariableName=meter_2  SampleTime=-1
  Ghi chỉ số 3 : ToWorkspace  VariableName=meter_3  SampleTime=-1
  Ghi chỉ số 4 : ToWorkspace  VariableName=meter_4  SampleTime=-1
  Ghi số mẫu hợp lệ : ToWorkspace  VariableName=valid_count  SampleTime=-1
  Mẫu hợp lệ : Subsystem
  Tính các chỉ số : Subsystem
  Tổng năng lượng : Subsystem
  SNR In : Outport
  SNR Out : Outport  Port=2
  Delta SNR : Outport  Port=3
  RMSE : Outport  Port=4
  wires:
  Mẫu hợp lệ/3(Output 3) -> Ghi số mẫu hợp lệ/1
  u_clean/1 -> Tổng năng lượng/1(In 1)
  u_noisy/1 -> Tổng năng lượng/2(In 2)
  u_denoised/1 -> Tổng năng lượng/3(In 3)
  Mẫu hợp lệ/1(Output 1) -> Tổng năng lượng/4(In 4)
  Tính các chỉ số/1(Đầu ra 1) -> SNR In/1, Ghi chỉ số 1/1
  Tính các chỉ số/2(Đầu ra 2) -> SNR Out/1, Ghi chỉ số 2/1
  Tính các chỉ số/3(Đầu ra 3) -> Delta SNR/1, Ghi chỉ số 3/1
  Tính các chỉ số/4(Đầu ra 4) -> Ghi chỉ số 4/1, RMSE/1
  Tổng năng lượng/1(Out 1) -> Tính các chỉ số/1(Input 1)
  Tổng năng lượng/2(Out 2) -> Tính các chỉ số/2(Input 2)
  Tổng năng lượng/3(Out 3) -> Tính các chỉ số/3(Input 3)
  Tổng năng lượng/4(Out 4) -> Tính các chỉ số/4(Input 4)
  Mẫu hợp lệ/2(Output 2) -> Tính các chỉ số/5(Input 5)

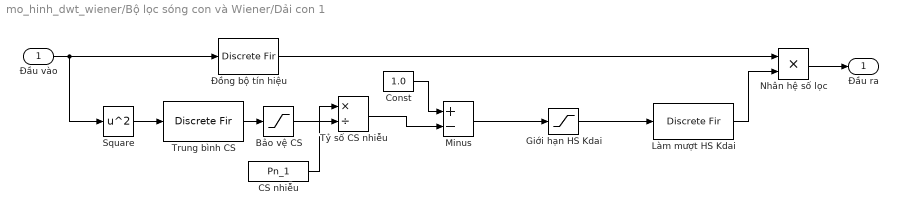
== system mo_hinh_dwt_wiener/Bộ lọc sóng con và Wiener/Dải con 1 ==
  Đầu vào : Inport
  Bảo vệ CS : Saturate  UpperLimit=inf  LowerLimit=realmin
  CS nhiễu : Constant  Value=Pn_1
  Const : Constant  Value=1.0
  Giới hạn HS Kdai : Saturate  UpperLimit=1.0  LowerLimit=Gain_Floor
  Làm mượt HS Kdai : DiscreteFir  Tag=WaveletDSP:sm_1  LoadFcn=dspblkCoreblockFVToolHelper(gcbh,'load');  Coefficients=ones(1,Sample_Count)/Sample_Count  InputProcessing=Columns as channels (frame based)  mask{Sample_Count=320}
      mask prompts: Sample_Count "Số mẫu cửa sổ (tự tính từ thiết lập bộ lọc)"
      mask help: Trung bình các mẫu trong cửa sổ. Chỉnh thời gian cửa sổ tại bộ lọc; không cần nhập dãy hệ số.
      mask init:
      | validateattributes(Sample_Count,{'double'},{'scalar','integer','finite','>=',1});
      settings: CopyFcn=dspblkCoreblockFVToolHelper(gcbh,'copy');  DeleteFcn=dspblkCoreblockFVToolHelper(gcbh,'close');  ModelCloseFcn=dspblkCoreblockFVToolHelper(gcbh,'close');  PreSaveFcn=dspblkCoreblockFVToolHelper(gcbh,'presave');  PostSaveFcn=dspblkCoreblockFVToolHelper(gcbh,'postsave');  CloseFcn=dspblkCoreblockFVToolHelper(gcbh,'close');
  Minus : Sum  Inputs=+-
  Nhân hệ số lọc : Product
  Square : Math  Operator=square
  Trung bình CS : DiscreteFir  Tag=WaveletDSP:pow_1  LoadFcn=dspblkCoreblockFVToolHelper(gcbh,'load');  Coefficients=ones(1,Sample_Count)/Sample_Count  InputProcessing=Columns as channels (frame based)  mask{Sample_Count=512}
      mask prompts: Sample_Count "Số mẫu cửa sổ (tự tính từ thiết lập bộ lọc)"
      mask help: Trung bình các mẫu trong cửa sổ. Chỉnh thời gian cửa sổ tại bộ lọc; không cần nhập dãy hệ số.
      mask init:
      | validateattributes(Sample_Count,{'double'},{'scalar','integer','finite','>=',1});
      settings: CopyFcn=dspblkCoreblockFVToolHelper(gcbh,'copy');  DeleteFcn=dspblkCoreblockFVToolHelper(gcbh,'close');  ModelCloseFcn=dspblkCoreblockFVToolHelper(gcbh,'close');  PreSaveFcn=dspblkCoreblockFVToolHelper(gcbh,'presave');  PostSaveFcn=dspblkCoreblockFVToolHelper(gcbh,'postsave');  CloseFcn=dspblkCoreblockFVToolHelper(gcbh,'close');
  Tỷ số CS nhiễu : Product  Inputs=*/
  Đồng bộ tín hiệu : DiscreteFir  Tag=WaveletDSP:sync_1  LoadFcn=dspblkCoreblockFVToolHelper(gcbh,'load');  Coefficients=[zeros(1,Sample_Count) 1]  InputProcessing=Columns as channels (frame based)  mask{Sample_Count=414}
      mask prompts: Sample_Count "Số mẫu đồng bộ (tự tính từ cấu trúc và thiết lập bộ lọc)"
      mask help: Đồng bộ tín hiệu theo số mẫu. Giá trị được tính tự động để giữ nguyên phép lọc; không cần nhập dãy hệ số.
      mask init:
      | validateattributes(Sample_Count,{'double'},{'scalar','integer','finite','>=',0});
      settings: CopyFcn=dspblkCoreblockFVToolHelper(gcbh,'copy');  DeleteFcn=dspblkCoreblockFVToolHelper(gcbh,'close');  ModelCloseFcn=dspblkCoreblockFVToolHelper(gcbh,'close');  PreSaveFcn=dspblkCoreblockFVToolHelper(gcbh,'presave');  PostSaveFcn=dspblkCoreblockFVToolHelper(gcbh,'postsave');  CloseFcn=dspblkCoreblockFVToolHelper(gcbh,'close');
  Đầu ra : Outport
  wires:
  Đầu vào/1 -> Đồng bộ tín hiệu/1, Square/1
  Square/1 -> Trung bình CS/1
  Trung bình CS/1 -> Bảo vệ CS/1
  CS nhiễu/1 -> Tỷ số CS nhiễu/1
  Bảo vệ CS/1 -> Tỷ số CS nhiễu/2
  Const/1 -> Minus/1
  Tỷ số CS nhiễu/1 -> Minus/2
  Minus/1 -> Giới hạn HS Kdai/1
  Giới hạn HS Kdai/1 -> Làm mượt HS Kdai/1
  Đồng bộ tín hiệu/1 -> Nhân hệ số lọc/1
  Làm mượt HS Kdai/1 -> Nhân hệ số lọc/2
  Nhân hệ số lọc/1 -> Đầu ra/1

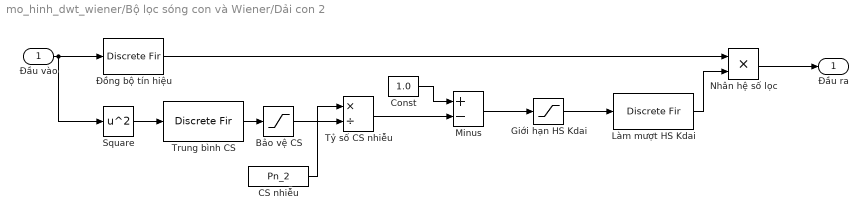
== system mo_hinh_dwt_wiener/Bộ lọc sóng con và Wiener/Dải con 2 ==
  Đầu vào : Inport
  Bảo vệ CS : Saturate  UpperLimit=inf  LowerLimit=realmin
  CS nhiễu : Constant  Value=Pn_2
  Const : Constant  Value=1.0
  Giới hạn HS Kdai : Saturate  UpperLimit=1.0  LowerLimit=Gain_Floor
  Làm mượt HS Kdai : DiscreteFir  Tag=WaveletDSP:sm_2  Coefficients=ones(1,Sample_Count)/Sample_Count  InputProcessing=Columns as channels (frame based)  mask{Sample_Count=160}
      mask prompts: Sample_Count "Số mẫu cửa sổ (tự tính từ thiết lập bộ lọc)"
      mask help: Trung bình các mẫu trong cửa sổ. Chỉnh thời gian cửa sổ tại bộ lọc; không cần nhập dãy hệ số.
      mask init:
      | validateattributes(Sample_Count,{'double'},{'scalar','integer','finite','>=',1});
  Minus : Sum  Inputs=+-
  Nhân hệ số lọc : Product
  Square : Math  Operator=square
  Trung bình CS : DiscreteFir  Tag=WaveletDSP:pow_2  Coefficients=ones(1,Sample_Count)/Sample_Count  InputProcessing=Columns as channels (frame based)  mask{Sample_Count=256}
      mask prompts: Sample_Count "Số mẫu cửa sổ (tự tính từ thiết lập bộ lọc)"
      mask help: Trung bình các mẫu trong cửa sổ. Chỉnh thời gian cửa sổ tại bộ lọc; không cần nhập dãy hệ số.
      mask init:
      | validateattributes(Sample_Count,{'double'},{'scalar','integer','finite','>=',1});
  Tỷ số CS nhiễu : Product  Inputs=*/
  Đồng bộ tín hiệu : DiscreteFir  Tag=WaveletDSP:sync_2  Coefficients=[zeros(1,Sample_Count) 1]  InputProcessing=Columns as channels (frame based)  mask{Sample_Count=206}
      mask prompts: Sample_Count "Số mẫu đồng bộ (tự tính từ cấu trúc và thiết lập bộ lọc)"
      mask help: Đồng bộ tín hiệu theo số mẫu. Giá trị được tính tự động để giữ nguyên phép lọc; không cần nhập dãy hệ số.
      mask init:
      | validateattributes(Sample_Count,{'double'},{'scalar','integer','finite','>=',0});
  Đầu ra : Outport
  wires:
  Đầu vào/1 -> Đồng bộ tín hiệu/1, Square/1
  Square/1 -> Trung bình CS/1
  Trung bình CS/1 -> Bảo vệ CS/1
  CS nhiễu/1 -> Tỷ số CS nhiễu/1
  Bảo vệ CS/1 -> Tỷ số CS nhiễu/2
  Const/1 -> Minus/1
  Tỷ số CS nhiễu/1 -> Minus/2
  Minus/1 -> Giới hạn HS Kdai/1
  Giới hạn HS Kdai/1 -> Làm mượt HS Kdai/1
  Đồng bộ tín hiệu/1 -> Nhân hệ số lọc/1
  Làm mượt HS Kdai/1 -> Nhân hệ số lọc/2
  Nhân hệ số lọc/1 -> Đầu ra/1

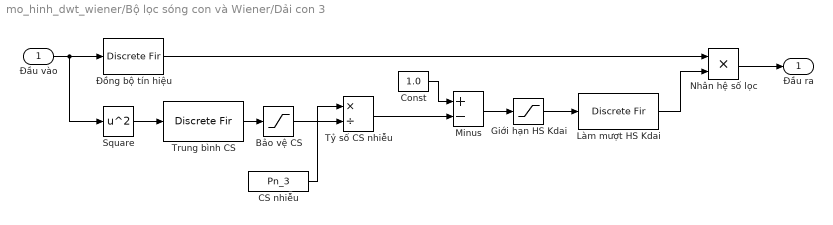
== system mo_hinh_dwt_wiener/Bộ lọc sóng con và Wiener/Dải con 3 ==
  Đầu vào : Inport
  Bảo vệ CS : Saturate  UpperLimit=inf  LowerLimit=realmin
  CS nhiễu : Constant  Value=Pn_3
  Const : Constant  Value=1.0
  Giới hạn HS Kdai : Saturate  UpperLimit=1.0  LowerLimit=Gain_Floor
  Làm mượt HS Kdai : DiscreteFir  Tag=WaveletDSP:sm_3  Coefficients=ones(1,Sample_Count)/Sample_Count  InputProcessing=Columns as channels (frame based)  mask{Sample_Count=80}
      mask prompts: Sample_Count "Số mẫu cửa sổ (tự tính từ thiết lập bộ lọc)"
      mask help: Trung bình các mẫu trong cửa sổ. Chỉnh thời gian cửa sổ tại bộ lọc; không cần nhập dãy hệ số.
      mask init:
      | validateattributes(Sample_Count,{'double'},{'scalar','integer','finite','>=',1});
  Minus : Sum  Inputs=+-
  Nhân hệ số lọc : Product
  Square : Math  Operator=square
  Trung bình CS : DiscreteFir  Tag=WaveletDSP:pow_3  Coefficients=ones(1,Sample_Count)/Sample_Count  InputProcessing=Columns as channels (frame based)  mask{Sample_Count=128}
      mask prompts: Sample_Count "Số mẫu cửa sổ (tự tính từ thiết lập bộ lọc)"
      mask help: Trung bình các mẫu trong cửa sổ. Chỉnh thời gian cửa sổ tại bộ lọc; không cần nhập dãy hệ số.
      mask init:
      | validateattributes(Sample_Count,{'double'},{'scalar','integer','finite','>=',1});
  Tỷ số CS nhiễu : Product  Inputs=*/
  Đồng bộ tín hiệu : DiscreteFir  Tag=WaveletDSP:sync_3  Coefficients=[zeros(1,Sample_Count) 1]  InputProcessing=Columns as channels (frame based)  mask{Sample_Count=102}
      mask prompts: Sample_Count "Số mẫu đồng bộ (tự tính từ cấu trúc và thiết lập bộ lọc)"
      mask help: Đồng bộ tín hiệu theo số mẫu. Giá trị được tính tự động để giữ nguyên phép lọc; không cần nhập dãy hệ số.
      mask init:
      | validateattributes(Sample_Count,{'double'},{'scalar','integer','finite','>=',0});
  Đầu ra : Outport
  wires:
  Đầu vào/1 -> Đồng bộ tín hiệu/1, Square/1
  Square/1 -> Trung bình CS/1
  Trung bình CS/1 -> Bảo vệ CS/1
  CS nhiễu/1 -> Tỷ số CS nhiễu/1
  Bảo vệ CS/1 -> Tỷ số CS nhiễu/2
  Const/1 -> Minus/1
  Tỷ số CS nhiễu/1 -> Minus/2
  Minus/1 -> Giới hạn HS Kdai/1
  Giới hạn HS Kdai/1 -> Làm mượt HS Kdai/1
  Đồng bộ tín hiệu/1 -> Nhân hệ số lọc/1
  Làm mượt HS Kdai/1 -> Nhân hệ số lọc/2
  Nhân hệ số lọc/1 -> Đầu ra/1

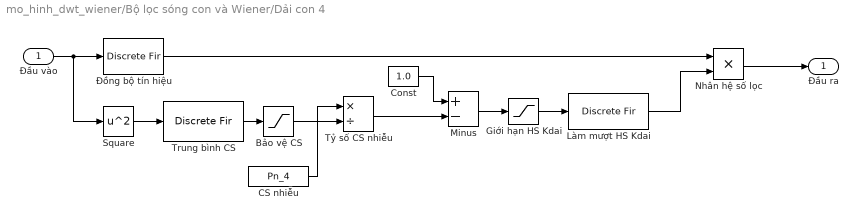
== system mo_hinh_dwt_wiener/Bộ lọc sóng con và Wiener/Dải con 4 ==
  Đầu vào : Inport
  Bảo vệ CS : Saturate  UpperLimit=inf  LowerLimit=realmin
  CS nhiễu : Constant  Value=Pn_4
  Const : Constant  Value=1.0
  Giới hạn HS Kdai : Saturate  UpperLimit=1.0  LowerLimit=Gain_Floor
  Làm mượt HS Kdai : DiscreteFir  Tag=WaveletDSP:sm_4  Coefficients=ones(1,Sample_Count)/Sample_Count  InputProcessing=Columns as channels (frame based)  mask{Sample_Count=40}
      mask prompts: Sample_Count "Số mẫu cửa sổ (tự tính từ thiết lập bộ lọc)"
      mask help: Trung bình các mẫu trong cửa sổ. Chỉnh thời gian cửa sổ tại bộ lọc; không cần nhập dãy hệ số.
      mask init:
      | validateattributes(Sample_Count,{'double'},{'scalar','integer','finite','>=',1});
  Minus : Sum  Inputs=+-
  Nhân hệ số lọc : Product
  Square : Math  Operator=square
  Trung bình CS : DiscreteFir  Tag=WaveletDSP:pow_4  Coefficients=ones(1,Sample_Count)/Sample_Count  InputProcessing=Columns as channels (frame based)  mask{Sample_Count=64}
      mask prompts: Sample_Count "Số mẫu cửa sổ (tự tính từ thiết lập bộ lọc)"
      mask help: Trung bình các mẫu trong cửa sổ. Chỉnh thời gian cửa sổ tại bộ lọc; không cần nhập dãy hệ số.
      mask init:
      | validateattributes(Sample_Count,{'double'},{'scalar','integer','finite','>=',1});
  Tỷ số CS nhiễu : Product  Inputs=*/
  Đồng bộ tín hiệu : DiscreteFir  Tag=WaveletDSP:sync_4  Coefficients=[zeros(1,Sample_Count) 1]  InputProcessing=Columns as channels (frame based)  mask{Sample_Count=50}
      mask prompts: Sample_Count "Số mẫu đồng bộ (tự tính từ cấu trúc và thiết lập bộ lọc)"
      mask help: Đồng bộ tín hiệu theo số mẫu. Giá trị được tính tự động để giữ nguyên phép lọc; không cần nhập dãy hệ số.
      mask init:
      | validateattributes(Sample_Count,{'double'},{'scalar','integer','finite','>=',0});
  Đầu ra : Outport
  wires:
  Đầu vào/1 -> Đồng bộ tín hiệu/1, Square/1
  Square/1 -> Trung bình CS/1
  Trung bình CS/1 -> Bảo vệ CS/1
  CS nhiễu/1 -> Tỷ số CS nhiễu/1
  Bảo vệ CS/1 -> Tỷ số CS nhiễu/2
  Const/1 -> Minus/1
  Tỷ số CS nhiễu/1 -> Minus/2
  Minus/1 -> Giới hạn HS Kdai/1
  Giới hạn HS Kdai/1 -> Làm mượt HS Kdai/1
  Đồng bộ tín hiệu/1 -> Nhân hệ số lọc/1
  Làm mượt HS Kdai/1 -> Nhân hệ số lọc/2
  Nhân hệ số lọc/1 -> Đầu ra/1

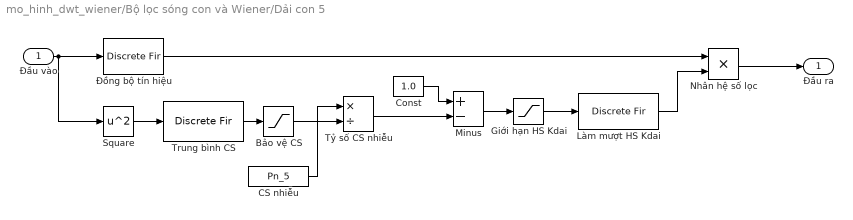
== system mo_hinh_dwt_wiener/Bộ lọc sóng con và Wiener/Dải con 5 ==
  Đầu vào : Inport
  Bảo vệ CS : Saturate  UpperLimit=inf  LowerLimit=realmin
  CS nhiễu : Constant  Value=Pn_5
  Const : Constant  Value=1.0
  Giới hạn HS Kdai : Saturate  UpperLimit=1.0  LowerLimit=Gain_Floor
  Làm mượt HS Kdai : DiscreteFir  Tag=WaveletDSP:sm_5  Coefficients=ones(1,Sample_Count)/Sample_Count  InputProcessing=Columns as channels (frame based)  mask{Sample_Count=20}
      mask prompts: Sample_Count "Số mẫu cửa sổ (tự tính từ thiết lập bộ lọc)"
      mask help: Trung bình các mẫu trong cửa sổ. Chỉnh thời gian cửa sổ tại bộ lọc; không cần nhập dãy hệ số.
      mask init:
      | validateattributes(Sample_Count,{'double'},{'scalar','integer','finite','>=',1});
  Minus : Sum  Inputs=+-
  Nhân hệ số lọc : Product
  Square : Math  Operator=square
  Trung bình CS : DiscreteFir  Tag=WaveletDSP:pow_5  Coefficients=ones(1,Sample_Count)/Sample_Count  InputProcessing=Columns as channels (frame based)  mask{Sample_Count=32}
      mask prompts: Sample_Count "Số mẫu cửa sổ (tự tính từ thiết lập bộ lọc)"
      mask help: Trung bình các mẫu trong cửa sổ. Chỉnh thời gian cửa sổ tại bộ lọc; không cần nhập dãy hệ số.
      mask init:
      | validateattributes(Sample_Count,{'double'},{'scalar','integer','finite','>=',1});
  Tỷ số CS nhiễu : Product  Inputs=*/
  Đồng bộ tín hiệu : DiscreteFir  Tag=WaveletDSP:sync_5  Coefficients=[zeros(1,Sample_Count) 1]  InputProcessing=Columns as channels (frame based)  mask{Sample_Count=24}
      mask prompts: Sample_Count "Số mẫu đồng bộ (tự tính từ cấu trúc và thiết lập bộ lọc)"
      mask help: Đồng bộ tín hiệu theo số mẫu. Giá trị được tính tự động để giữ nguyên phép lọc; không cần nhập dãy hệ số.
      mask init:
      | validateattributes(Sample_Count,{'double'},{'scalar','integer','finite','>=',0});
  Đầu ra : Outport
  wires:
  Đầu vào/1 -> Đồng bộ tín hiệu/1, Square/1
  Square/1 -> Trung bình CS/1
  Trung bình CS/1 -> Bảo vệ CS/1
  CS nhiễu/1 -> Tỷ số CS nhiễu/1
  Bảo vệ CS/1 -> Tỷ số CS nhiễu/2
  Const/1 -> Minus/1
  Tỷ số CS nhiễu/1 -> Minus/2
  Minus/1 -> Giới hạn HS Kdai/1
  Giới hạn HS Kdai/1 -> Làm mượt HS Kdai/1
  Đồng bộ tín hiệu/1 -> Nhân hệ số lọc/1
  Làm mượt HS Kdai/1 -> Nhân hệ số lọc/2
  Nhân hệ số lọc/1 -> Đầu ra/1

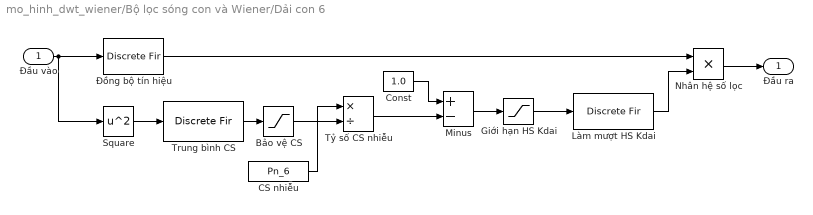
== system mo_hinh_dwt_wiener/Bộ lọc sóng con và Wiener/Dải con 6 ==
  Đầu vào : Inport
  Bảo vệ CS : Saturate  UpperLimit=inf  LowerLimit=realmin
  CS nhiễu : Constant  Value=Pn_6
  Const : Constant  Value=1.0
  Giới hạn HS Kdai : Saturate  UpperLimit=1.0  LowerLimit=Gain_Floor
  Làm mượt HS Kdai : DiscreteFir  Tag=WaveletDSP:sm_6  Coefficients=ones(1,Sample_Count)/Sample_Count  InputProcessing=Columns as channels (frame based)  mask{Sample_Count=10}
      mask prompts: Sample_Count "Số mẫu cửa sổ (tự tính từ thiết lập bộ lọc)"
      mask help: Trung bình các mẫu trong cửa sổ. Chỉnh thời gian cửa sổ tại bộ lọc; không cần nhập dãy hệ số.
      mask init:
      | validateattributes(Sample_Count,{'double'},{'scalar','integer','finite','>=',1});
  Minus : Sum  Inputs=+-
  Nhân hệ số lọc : Product
  Square : Math  Operator=square
  Trung bình CS : DiscreteFir  Tag=WaveletDSP:pow_6  Coefficients=ones(1,Sample_Count)/Sample_Count  InputProcessing=Columns as channels (frame based)  mask{Sample_Count=16}
      mask prompts: Sample_Count "Số mẫu cửa sổ (tự tính từ thiết lập bộ lọc)"
      mask help: Trung bình các mẫu trong cửa sổ. Chỉnh thời gian cửa sổ tại bộ lọc; không cần nhập dãy hệ số.
      mask init:
      | validateattributes(Sample_Count,{'double'},{'scalar','integer','finite','>=',1});
  Tỷ số CS nhiễu : Product  Inputs=*/
  Đồng bộ tín hiệu : DiscreteFir  Tag=WaveletDSP:sync_6  Coefficients=[zeros(1,Sample_Count) 1]  InputProcessing=Columns as channels (frame based)  mask{Sample_Count=11}
      mask prompts: Sample_Count "Số mẫu đồng bộ (tự tính từ cấu trúc và thiết lập bộ lọc)"
      mask help: Đồng bộ tín hiệu theo số mẫu. Giá trị được tính tự động để giữ nguyên phép lọc; không cần nhập dãy hệ số.
      mask init:
      | validateattributes(Sample_Count,{'double'},{'scalar','integer','finite','>=',0});
  Đầu ra : Outport
  wires:
  Đầu vào/1 -> Đồng bộ tín hiệu/1, Square/1
  Square/1 -> Trung bình CS/1
  Trung bình CS/1 -> Bảo vệ CS/1
  CS nhiễu/1 -> Tỷ số CS nhiễu/1
  Bảo vệ CS/1 -> Tỷ số CS nhiễu/2
  Const/1 -> Minus/1
  Tỷ số CS nhiễu/1 -> Minus/2
  Minus/1 -> Giới hạn HS Kdai/1
  Giới hạn HS Kdai/1 -> Làm mượt HS Kdai/1
  Đồng bộ tín hiệu/1 -> Nhân hệ số lọc/1
  Làm mượt HS Kdai/1 -> Nhân hệ số lọc/2
  Nhân hệ số lọc/1 -> Đầu ra/1
